simulink library "Contact_Forces_Lib"  (R2025a)
settings: Solver=ode45  StartTime=0.0  StopTime=10.0  RelTol=1e-3  EnableMultiTasking=on
undefined symbols (not defined in the file or in its folder): b_contact, custom_param_1, custom_param_2, Extr_Data_Ring, k_contact, l_cone, length_cylinder, length_tube, mu_kinetic, mu_static, pen_exponent, pen_full_damp_F, rad_s_cone, radius_cylinder, radius_tube, v_thr, X, Y, Z
libraries: nesl_utility x197, sm_lib x115, $bdroot x72, simulink x20, fl_lib x4
(part 8 of 12)

== system Contact_Forces_Lib/3D/Sphere to Tube Force Enabled/Demux ==
  Frc : Inport
  Demux : Demux  Outputs=8
  Demux1 : Demux  Outputs=3
  Scope : Scope  NumInputPorts=6
      settings: ActiveDisplayYMinimum=-4577.1518  ActiveDisplayYMaximum=26358.32622
  Simulink-PS Converter{,1..7} (8 alike) : nesl_utility/Simulink-PS Converter  PhysicalDomain=network_engine_domain  SubClassName=ps_input  LeftPortType=input  RightPortType=output  PseudoPeriodic=off  Frequencies=[]  NoiseDistribution=none  NoiseParameters=[]  Unit=1  AffineConversion=off  FilteringAndDerivatives=zero  SimscapeFilterOrder=1  InputFilterTimeConstant=0.005  UdotUserProvided=1
  FxF : PMIOPort  Side=Right
  FyF : PMIOPort  Port=2  Side=Right
  FzF : PMIOPort  Port=3  Side=Right
  TF : PMIOPort  Port=4  Side=Right
  FxB : PMIOPort  Port=5  Side=Right
  FyB : PMIOPort  Port=6  Side=Right
  FzB : PMIOPort  Port=7  Side=Right
  TB : PMIOPort  Port=8  Side=Right
  wires:
  Demux1/3 -> Scope/6  "Tz"
  Demux1/2 -> Scope/5  "Ty"
  Demux1/1 -> Scope/4  "Tx"
  Demux/5 -> Simulink-PS Converter3/1, Scope/1  "Fx"
  Demux/6 -> Simulink-PS Converter4/1, Scope/2  "Fy"
  Demux/8 -> Simulink-PS Converter5/1, Demux1/1
  Demux/7 -> Simulink-PS Converter7/1, Scope/3  "Fz"
  Demux/3 -> Simulink-PS Converter6/1  "Fz"
  Demux/4 -> Simulink-PS Converter2/1
  Demux/2 -> Simulink-PS Converter1/1  "Fy"
  Demux/1 -> Simulink-PS Converter/1  "Fx"
  Frc/1 -> Demux/1
  connections:
  Simulink-PS Converter7/RConn1 -- FzB/RConn1
  Simulink-PS Converter6/RConn1 -- FzF/RConn1
  Simulink-PS Converter1/RConn1 -- FyF/RConn1
  Simulink-PS Converter/RConn1 -- FxF/RConn1
  Simulink-PS Converter5/RConn1 -- TB/RConn1
  Simulink-PS Converter3/RConn1 -- FxB/RConn1
  Simulink-PS Converter4/RConn1 -- FyB/RConn1
  Simulink-PS Converter2/RConn1 -- TF/RConn1

== system Contact_Forces_Lib/3D/Sphere to Tube Force Enabled/Forces ==
  z : Inport
  rad : Inport  Port=2
  vrad : Inport  Port=3
  azm : Inport  Port=4
  vazm : Inport  Port=5
  wzf : Inport  Port=6
  R : Inport  Port=7
  vzf : Inport  Port=8
  wxf : Inport  Port=9
  wyf : Inport  Port=10
  Action Port : ActionPort
  Bus Creator : BusCreator  Inputs=6
  Calculate Penetration : Subsystem
  Ff : Subsystem
  Fn : Subsystem
  Force Law : $bdroot/Force Law  SystemSampleTime=-1  LabelModeActiveChoice=Linear  VariantActivationTime=update diagram  EmptyChoice=off  PassThrough=off  PassThroughVariantControl=(default)  EmptyChoiceVariantControl=(default)  AllowFlexibleInterface=on  Latency=0  AutoFrameSizeCalculation=off
  Gain : Gain  Gain=-1
  Mux : Mux  Inputs=8
  Product : Product
  Sum : Subsystem
  Sum1 : Sum  Inputs=+-
  Frc : Outport  VectorParamsAs1DForOutWhenUnconnected=off
  Out : Outport  Port=2  InitialOutput=[0]  VectorParamsAs1DForOutWhenUnconnected=off
  wires:
  wyf/1 -> Ff/11(wyf)
  wxf/1 -> Ff/10(wxf)
  Gain/1 -> Ff/1(Fn)
  vzf/1 -> Ff/9(vzf)
  wzf/1 -> Ff/6(wzf)
  vazm/1 -> Ff/5(vazm)
  Sum/8(TB) -> Mux/8
  Sum/7(FzB) -> Mux/7
  Ff/9(Ff) -> Bus Creator/6  "Friction Force"
  Sum/3(FzF) -> Mux/3
  Sum/6(FyB) -> Mux/6
  Sum/5(FxB) -> Mux/5
  Sum/4(TzF) -> Mux/4
  Mux/1 -> Frc/1
  Sum/1(FxF) -> Mux/1
  Sum/2(FyF) -> Mux/2
  azm/1 -> Ff/4(azm), Fn/4(azm)
  R/1 -> Ff/3(R), Fn/3(R)
  Sum1/1 -> Product/2
  Force Law/2 -> Sum1/2, Bus Creator/3  "Damp Force"
  Calculate Penetration/1(sign) -> Product/1
  Calculate Penetration/2(Pen) -> Force Law/1, Bus Creator/2, Ff/7(Pen)  "Penetration"
  Product/1 -> Gain/1, Fn/1(Fn), Bus Creator/5  "Normal Force"
  rad/1 -> Calculate Penetration/1(rad), Ff/8(rad)
  vrad/1 -> Calculate Penetration/2(vrad)
  Calculate Penetration/3(Pen Vel) -> Force Law/2, Bus Creator/1  "Penetration Vel"
  Force Law/1 -> Sum1/1, Bus Creator/4  "Spr Force"
  Bus Creator/1 -> Out/1
  z/1 -> Fn/2(z), Ff/2(z)
  Fn/2(FySphF) -> Sum/2(FnySphF)
  Fn/1(FxSphF) -> Sum/1(FnxSphF)
  Fn/3(FZSphF) -> Sum/3(FnzSphF)
  Fn/4(FxTubB) -> Sum/4(FnxTubB)
  Fn/5(FyTubB) -> Sum/5(FnyTubB)
  Fn/6(TxTubB) -> Sum/6(TnxTubB)
  Fn/7(TyTubB) -> Sum/7(TnyTubB)
  Ff/1(FxSphF) -> Sum/8(FfxSphF)
  Ff/2(FySohF) -> Sum/9(FfySphF)
  Ff/3(FzSphF) -> Sum/10(FfzSphF)
  Ff/4(FxTubB) -> Sum/11(FfxTubB)
  Ff/5(FyTubB) -> Sum/12(FfyTubB)
  Ff/6(FzTubB) -> Sum/13(FfzTubB)
  Ff/7(TSphF) -> Sum/14(TzSphF)
  Ff/8(TTubB) -> Sum/15(TTubB)

== system Contact_Forces_Lib/3D/Sphere to Tube Force Enabled/No Force ==
  Action Port : ActionPort
  Zeros : Constant  Value=[0 0 0 0 0 0 0 0 0 0 0 0]  SampleTime=0
  F : Outport  InitialOutput=[0]  VectorParamsAs1DForOutWhenUnconnected=off
  wires:
  Zeros/1 -> F/1

== system Contact_Forces_Lib/3D/Sphere to Tube Force Enabled/Sensing ==
  In : Inport
  Bus Selector : BusSelector  OutputSignals=wz
  In or Out : Subsystem
  PS-Simulink Converter{1..4,6..11} (10 alike) : nesl_utility/PS-Simulink Converter  PhysicalDomain=network_engine_domain  SubClassName=ps_output  LeftPortType=input  RightPortType=output  PseudoPeriodic=off  Frequencies=[]  VectorFormat=1-D array  Unit=1  AffineConversion=off
  Product : Product
  Rotation F in B : Gain  Gain=1/radius_sphere
  Sum : Sum  Inputs=|+-
  Transform Sensor Base : sm_lib/Frames and Transforms/Transform Sensor  MeasurementFrame=Base  RotationSequence=XYX  SenseAngle=off  SenseAxis=off  SenseQ=off  SenseR=on  SenseRotationSequence=off  SenseOmegaX=on  SenseOmegaY=on  SenseOmegaZ=on  SenseOmega=off  SenseQDot=off  SenseRDot=off  SenseRotationSequenceDot=off  SenseAlphaX=off  SenseAlphaY=off  SenseAlphaZ=off  SenseAlpha=off  SenseQDDot=off  SenseRDDot=off  SenseX=on  SenseY=on  SenseZ=on  SenseXYZ=off  SenseRad=off  SenseAzim=off  SenseDist=off  SenseInc=off  SenseXDot=on  SenseYDot=on  SenseZDot=on  SenseXYZDot=off  SenseRadDot=off  SenseAzimDot=off  SenseDistDot=off  SenseIncDot=off  SenseXDDot=off  SenseYDDot=off  SenseZDDot=off  SenseXYZDDot=off  SenseRadDDot=off  SenseAzimDDot=off  SenseDistDDot=off  SenseIncDDot=off
  rad_azm_cal : Subsystem
  F : PMIOPort  Side=Left
  B : PMIOPort  Port=2  Side=Left
  z : Outport  VectorParamsAs1DForOutWhenUnconnected=off
  rad : Outport  Port=2  VectorParamsAs1DForOutWhenUnconnected=off
  vrad : Outport  Port=3  VectorParamsAs1DForOutWhenUnconnected=off
  azm : Outport  Port=4  VectorParamsAs1DForOutWhenUnconnected=off
  vazm : Outport  Port=5  VectorParamsAs1DForOutWhenUnconnected=off
  wzf : Outport  Port=6  VectorParamsAs1DForOutWhenUnconnected=off
  R : Outport  Port=7  VectorParamsAs1DForOutWhenUnconnected=off
  vzf : Outport  Port=8  VectorParamsAs1DForOutWhenUnconnected=off
  wxf : Outport  Port=9  VectorParamsAs1DForOutWhenUnconnected=off
  wyf : Outport  Port=10  VectorParamsAs1DForOutWhenUnconnected=off
  wires:
  Sum/1 -> wzf/1
  rad_azm_cal/1(rad) -> In or Out/1(rad), rad/1
  Bus Selector/1 -> Rotation F in B/1  "<wz>"
  Product/1 -> Sum/2
  In/1 -> Bus Selector/1
  PS-Simulink Converter4/1 -> wyf/1
  PS-Simulink Converter3/1 -> wxf/1
  PS-Simulink Converter2/1 -> Sum/1
  PS-Simulink Converter1/1 -> vzf/1
  PS-Simulink Converter6/1 -> R/1
  rad_azm_cal/4(azmv) -> vazm/1
  rad_azm_cal/3(radv) -> vrad/1
  rad_azm_cal/2(azm) -> azm/1
  PS-Simulink Converter11/1 -> rad_azm_cal/4(Ydot)
  PS-Simulink Converter10/1 -> rad_azm_cal/3(Xdot)
  PS-Simulink Converter9/1 -> rad_azm_cal/2(Y)
  PS-Simulink Converter8/1 -> rad_azm_cal/1(X)
  PS-Simulink Converter7/1 -> z/1
  In or Out/1(factor) -> Product/2
  Rotation F in B/1 -> Product/1
  connections:
  PS-Simulink Converter2/LConn1 -- Transform Sensor Base/RConn5
  PS-Simulink Converter4/LConn1 -- Transform Sensor Base/RConn4
  Transform Sensor Base/RConn11 -- PS-Simulink Converter1/LConn1
  Transform Sensor Base/RConn10 -- PS-Simulink Converter11/LConn1
  Transform Sensor Base/RConn9 -- PS-Simulink Converter10/LConn1
  Transform Sensor Base/RConn8 -- PS-Simulink Converter7/LConn1
  Transform Sensor Base/RConn7 -- PS-Simulink Converter9/LConn1
  PS-Simulink Converter8/LConn1 -- Transform Sensor Base/RConn6
  PS-Simulink Converter3/LConn1 -- Transform Sensor Base/RConn3
  PS-Simulink Converter6/LConn1 -- Transform Sensor Base/RConn2
  Transform Sensor Base/LConn1 -- B/RConn1
  Transform Sensor Base/RConn1 -- F/RConn1

== system Contact_Forces_Lib/3D/Sphere to Tube Force Enabled/Set Output ==
  Frc : Inport
  En : Inport  Port=2
  FrameSep : Inport  Port=3
  Bus Creator : BusCreator  Inputs=7
  Bus Selector : BusSelector  OutputSignals=Normal Force,Friction Force,Penetration,Penetration Vel,Spr Force,Damp Force
  Demux : Demux  Outputs=6
  Mux : Mux  Inputs=6
  Product : Product
  Out : Outport  VectorParamsAs1DForOutWhenUnconnected=off
  wires:
  Bus Selector/2 -> Mux/2  "<Friction Force>"
  Bus Selector/4 -> Mux/4  "<Penetration Vel>"
  Bus Selector/6 -> Mux/6  "<Damp Force>"
  Bus Selector/3 -> Mux/3  "<Penetration>"
  Bus Creator/1 -> Out/1
  Bus Selector/1 -> Mux/1  "<Normal Force>"
  Bus Selector/5 -> Mux/5  "<Spr Force>"
  Frc/1 -> Bus Selector/1
  FrameSep/1 -> Bus Creator/7
  Mux/1 -> Product/2
  En/1 -> Product/1
  Product/1 -> Demux/1
  Demux/1 -> Bus Creator/1  "Normal Force"
  Demux/2 -> Bus Creator/2  "Friction Force"
  Demux/4 -> Bus Creator/4  "Penetration Vel"
  Demux/5 -> Bus Creator/5  "Spr Force"
  Demux/6 -> Bus Creator/6  "Damp Force"
  Demux/3 -> Bus Creator/3  "Penetration"

== system Contact_Forces_Lib/Force Law/Nonlinear/Smoothstep ==
  In1 : Inport
  Clamp : Saturate  UpperLimit=step_finish  LowerLimit=step_start
  Constant : Constant  Value=3
  Divide : Product  Inputs=*/
  Divide1 : Product  Inputs=****
  Gain : Gain  Gain=2
  Subtract : Sum  Inputs=+-
  Subtract1 : Sum  Inputs=-+
  Subtract2 : Sum
  Subtract3 : Sum  Inputs=+-
  Subtract4 : Sum  Inputs=+-
  max out : Constant  Value=max_out
  min out : Constant  Value=min_out
  step finish : Constant  Value=step_finish
  step start : Constant  Value=step_start
  Out1 : Outport  VectorParamsAs1DForOutWhenUnconnected=off
  wires:
  Subtract3/1 -> Divide1/4
  Subtract4/1 -> Divide1/1
  Gain/1 -> Subtract4/2
  Divide1/1 -> Subtract2/1
  step finish/1 -> Subtract1/2
  Clamp/1 -> Subtract/1
  max out/1 -> Subtract3/1
  min out/1 -> Subtract3/2, Subtract2/2
  Constant/1 -> Subtract4/1
  Subtract2/1 -> Out1/1
  Subtract/1 -> Divide/1
  Divide/1 -> Divide1/3, Divide1/2, Gain/1
  Subtract1/1 -> Divide/2
  In1/1 -> Clamp/1
  step start/1 -> Subtract/2, Subtract1/1

== system Contact_Forces_Lib/Friction Utilities/Stick-Slip Friction 1D/Lag Filter ==
  In : Inport
  Gain : Gain  Gain=1/b
  Integrator : Integrator  InitialCondition=x_initial
  Sum : Sum  Inputs=|+-  InputSameDT=on  SaturateOnIntegerOverflow=on  OutDataTypeStr=Inherit: Same as first input
  Out : Outport  VectorParamsAs1DForOutWhenUnconnected=off
  wires:
  Gain/1 -> Out/1, Sum/2
  Integrator/1 -> Gain/1
  In/1 -> Sum/1
  Sum/1 -> Integrator/1

== system Contact_Forces_Lib/Friction Utilities/Utilities/Product ==
  note: 1) Only subsystems can be added as variant choices at this level
      | 2) Blocks cannot be connected at this level as connectivity is
      | automatically determined at simulation, based on the active variant
  FcConst : Subsystem  VariantControl=FcConst
  FcVect : Subsystem  VariantControl=FcVect
  Fc : PMIOPort  Side=Right
  v : PMIOPort  Port=2  Side=Right

== system Contact_Forces_Lib/2D/Circle to Circle Force/Ff/Calculate vRel at CP  ==
  rad : Inport
  Pen : Inport  Port=2
  wz : Inport  Port=3
  vazm : Inport  Port=4
  Follower Radius : Constant  Value=cirF_rad
  Midpt Pen : Gain  Gain=0.5
  Product5 : Product
  Product6 : Product
  Sum{3,5..7} (4 alike) : Sum  Inputs=+-
  vRelCP : Outport  VectorParamsAs1DForOutWhenUnconnected=off
  rCirFtoCP : Outport  Port=2  VectorParamsAs1DForOutWhenUnconnected=off
  rCirBtoCP : Outport  Port=3  VectorParamsAs1DForOutWhenUnconnected=off
  wires:
  Follower Radius/1 -> Sum3/1
  Midpt Pen/1 -> Sum3/2
  Pen/1 -> Midpt Pen/1
  rad/1 -> Sum5/1
  Sum3/1 -> rCirFtoCP/1, Sum5/2, Product6/2
  vazm/1 -> Product5/1, Sum6/2
  Sum5/1 -> rCirBtoCP/1, Product5/2
  wz/1 -> Sum6/1
  Sum6/1 -> Product6/1
  Product5/1 -> Sum7/1
  Product6/1 -> Sum7/2
  Sum7/1 -> vRelCP/1

== system Contact_Forces_Lib/2D/Circle to Circle Force/Ff/Resolve Ff ==
  note: Resolve Friction Force in
      | Circle F reference frame
  note: Resolve Friction Force in
      | Circle B reference frame
  Ff : Inport
  R : Inport  Port=2
  azm : Inport  Port=3
  rCirFtoCP : Inport  Port=4
  rCirBtoCP : Inport  Port=5
  Ff in CirB : Subsystem
  Ff in CirF : Subsystem
  Tz : Subsystem
  FxCirB : Outport  VectorParamsAs1DForOutWhenUnconnected=off
  FyCirB : Outport  Port=2  VectorParamsAs1DForOutWhenUnconnected=off
  FyCirF : Outport  Port=3  VectorParamsAs1DForOutWhenUnconnected=off
  FxCirF : Outport  Port=4  VectorParamsAs1DForOutWhenUnconnected=off
  TzCirF : Outport  Port=5  VectorParamsAs1DForOutWhenUnconnected=off
  TzCirB : Outport  Port=6  VectorParamsAs1DForOutWhenUnconnected=off
  wires:
  Ff in CirF/2(FxCirF) -> FxCirF/1
  Ff in CirF/1(FyCirF) -> FyCirF/1
  R/1 -> Ff in CirF/1(R)
  azm/1 -> Ff in CirB/2(azm)
  Ff in CirB/2(FyCirB) -> Ff in CirF/3(FyCirB), FyCirB/1
  Ff in CirB/1(FxCirB) -> Ff in CirF/2(FxCirB), FxCirB/1
  Tz/2(TzF) -> TzCirF/1
  Tz/1(TzB) -> TzCirB/1
  Ff/1 -> Ff in CirB/1(Ff), Tz/3(Ff)
  rCirFtoCP/1 -> Tz/1(rCirFtoCP)
  rCirBtoCP/1 -> Tz/2(rCirBtoCP)

== system Contact_Forces_Lib/2D/Circle to Circle Force/Fn/Fn in CirB ==
  Fn : Inport
  azm : Inport  Port=2
  Divide1 : Product  Inputs=**
  Divide2 : Product  Inputs=**
  Gain2 : Gain  Gain=-1
  cos : Trigonometry  Operator=cos
  deg2rad : Gain  Gain=pi/180
  sin : Trigonometry
  FxCirB : Outport  VectorParamsAs1DForOutWhenUnconnected=off
  FyCirB : Outport  Port=2  VectorParamsAs1DForOutWhenUnconnected=off
  wires:
  azm/1 -> deg2rad/1
  Fn/1 -> Gain2/1
  Divide2/1 -> FyCirB/1  "Fy Cir"
  Divide1/1 -> FxCirB/1
  cos/1 -> Divide1/2
  sin/1 -> Divide2/2
  deg2rad/1 -> sin/1, cos/1
  Gain2/1 -> Divide2/1, Divide1/1

== system Contact_Forces_Lib/2D/Circle to Circle Force/Fn/Fn in CirF ==
  R : Inport
  FxCirB : Inport  Port=2
  FyCirB : Inport  Port=3
  Demux : Demux  Outputs=2
  Divide3 : Product  Inputs=**  Multiplication=Matrix(*)
  Gain : Gain  Gain=-1
  Mux1 : Mux  Inputs=2
  FyCirF : Outport  VectorParamsAs1DForOutWhenUnconnected=off
  FxCirF : Outport  Port=2  VectorParamsAs1DForOutWhenUnconnected=off
  wires:
  FxCirB/1 -> Mux1/2
  FyCirB/1 -> Mux1/1
  R/1 -> Divide3/1
  Divide3/1 -> Gain/1
  Mux1/1 -> Divide3/2
  Gain/1 -> Demux/1
  Demux/1 -> FyCirF/1
  Demux/2 -> FxCirF/1

== system Contact_Forces_Lib/2D/Circle to Circle Force Enabled/Ff/Calculate vRel at CP  ==
  rad : Inport
  Pen : Inport  Port=2
  wz : Inport  Port=3
  vazm : Inport  Port=4
  Follower Radius : Constant  Value=cirF_rad
  Midpt Pen : Gain  Gain=0.5
  Product5 : Product
  Product6 : Product
  Sum{3,5..7} (4 alike) : Sum  Inputs=+-
  vRelCP : Outport  VectorParamsAs1DForOutWhenUnconnected=off
  rCirFtoCP : Outport  Port=2  VectorParamsAs1DForOutWhenUnconnected=off
  rCirBtoCP : Outport  Port=3  VectorParamsAs1DForOutWhenUnconnected=off
  wires:
  Sum7/1 -> vRelCP/1
  Product6/1 -> Sum7/2
  Product5/1 -> Sum7/1
  Sum6/1 -> Product6/1
  wz/1 -> Sum6/1
  Sum5/1 -> Product5/2, rCirBtoCP/1
  vazm/1 -> Sum6/2, Product5/1
  Sum3/1 -> Product6/2, Sum5/2, rCirFtoCP/1
  rad/1 -> Sum5/1
  Pen/1 -> Midpt Pen/1
  Midpt Pen/1 -> Sum3/2
  Follower Radius/1 -> Sum3/1

== system Contact_Forces_Lib/2D/Circle to Circle Force Enabled/Ff/Resolve Ff ==
  note: Resolve Friction Force in
      | Circle B reference frame
  note: Resolve Friction Force in
      | Circle F reference frame
  Ff : Inport
  R : Inport  Port=2
  azm : Inport  Port=3
  rCirFtoCP : Inport  Port=4
  rCirBtoCP : Inport  Port=5
  Ff in CirB : Subsystem
  Ff in CirF : Subsystem
  Tz : Subsystem
  FxCirB : Outport  VectorParamsAs1DForOutWhenUnconnected=off
  FyCirB : Outport  Port=2  VectorParamsAs1DForOutWhenUnconnected=off
  FyCirF : Outport  Port=3  VectorParamsAs1DForOutWhenUnconnected=off
  FxCirF : Outport  Port=4  VectorParamsAs1DForOutWhenUnconnected=off
  TzCirF : Outport  Port=5  VectorParamsAs1DForOutWhenUnconnected=off
  TzCirB : Outport  Port=6  VectorParamsAs1DForOutWhenUnconnected=off
  wires:
  rCirBtoCP/1 -> Tz/2(rCirBtoCP)
  rCirFtoCP/1 -> Tz/1(rCirFtoCP)
  Ff/1 -> Tz/3(Ff), Ff in CirB/1(Ff)
  Tz/1(TzB) -> TzCirB/1
  Tz/2(TzF) -> TzCirF/1
  Ff in CirB/1(FxCirB) -> FxCirB/1, Ff in CirF/2(FxCirB)
  Ff in CirB/2(FyCirB) -> FyCirB/1, Ff in CirF/3(FyCirB)
  azm/1 -> Ff in CirB/2(azm)
  R/1 -> Ff in CirF/1(R)
  Ff in CirF/1(FyCirF) -> FyCirF/1
  Ff in CirF/2(FxCirF) -> FxCirF/1

== system Contact_Forces_Lib/2D/Circle to Circle Force Enabled/Fn/Fn in CirB ==
  Fn : Inport
  azm : Inport  Port=2
  Divide1 : Product  Inputs=**
  Divide2 : Product  Inputs=**
  Gain2 : Gain  Gain=-1
  cos : Trigonometry  Operator=cos
  deg2rad : Gain  Gain=pi/180
  sin : Trigonometry
  FxCirB : Outport  VectorParamsAs1DForOutWhenUnconnected=off
  FyCirB : Outport  Port=2  VectorParamsAs1DForOutWhenUnconnected=off
  wires:
  Gain2/1 -> Divide1/1, Divide2/1
  deg2rad/1 -> cos/1, sin/1
  sin/1 -> Divide2/2
  cos/1 -> Divide1/2
  Divide1/1 -> FxCirB/1
  Divide2/1 -> FyCirB/1  "Fy Cir"
  Fn/1 -> Gain2/1
  azm/1 -> deg2rad/1

== system Contact_Forces_Lib/2D/Circle to Circle Force Enabled/Fn/Fn in CirF ==
  R : Inport
  FxCirB : Inport  Port=2
  FyCirB : Inport  Port=3
  Demux : Demux  Outputs=2
  Divide3 : Product  Inputs=**  Multiplication=Matrix(*)
  Gain : Gain  Gain=-1
  Mux1 : Mux  Inputs=2
  FyCirF : Outport  VectorParamsAs1DForOutWhenUnconnected=off
  FxCirF : Outport  Port=2  VectorParamsAs1DForOutWhenUnconnected=off
  wires:
  Demux/2 -> FxCirF/1
  Demux/1 -> FyCirF/1
  Gain/1 -> Demux/1
  Mux1/1 -> Divide3/2
  Divide3/1 -> Gain/1
  R/1 -> Divide3/1
  FyCirB/1 -> Mux1/1
  FxCirB/1 -> Mux1/2

== system Contact_Forces_Lib/2D/Circle to Finite Line Force/Forces/Resolve Forces ==
  note: For circle, uses forces as calculated.
      | For line, force must be applied at CG.
      |        Apply torque corresponding to equivalent couple.
  Moment arm : Inport
  Pos Cmp : Inport  Port=2
  X Sep : Inport  Port=3
  Spr Force Mag : Inport  Port=4
  Damp Force Mag : Inport  Port=5
  Vel Cmp : Inport  Port=6
  Unit Vector : Inport  Port=7
  vy : Inport  Port=8
  wz : Inport  Port=9
  Divide4 : Product  Inputs=**
  FnCir : Subsystem
  FnLin : Subsystem
  Friction : Subsystem
  Gain : Gain  Gain=-1
  Product : Product  RndMeth=Zero
  Product1 : Product  RndMeth=Zero
  Sum{,1..4} (5 alike) : Sum
  Fx Cir : Outport  VectorParamsAs1DForOutWhenUnconnected=off
  Fy Cir : Outport  Port=2  VectorParamsAs1DForOutWhenUnconnected=off
  Tz Cir : Outport  Port=3  VectorParamsAs1DForOutWhenUnconnected=off
  Fx Lin : Outport  Port=4  VectorParamsAs1DForOutWhenUnconnected=off
  Fy Lin : Outport  Port=5  VectorParamsAs1DForOutWhenUnconnected=off
  Tz Lin : Outport  Port=6  VectorParamsAs1DForOutWhenUnconnected=off
  Fn : Outport  Port=7  VectorParamsAs1DForOutWhenUnconnected=off
  Ff : Outport  Port=8  VectorParamsAs1DForOutWhenUnconnected=off
  wires:
  X Sep/1 -> Friction/3(X Sep)
  Friction/5(TzCir) -> Tz Cir/1
  Sum1/1 -> Friction/2(Fn), FnCir/2(Fn), Divide4/1, Fn/1, FnLin/1(Fn)
  Sum2/1 -> Fx Cir/1
  Sum3/1 -> Fy Cir/1
  Sum4/1 -> Fy Lin/1
  FnLin/1(FxLin) -> Fx Lin/1
  Friction/3(FyLin) -> Sum4/1
  FnLin/2(FyLin) -> Sum4/2
  Friction/2(FyCir) -> Sum3/2
  FnCir/2(FyCir) -> Sum3/1
  FnCir/1(FxCir) -> Sum2/1
  Friction/1(FxCir) -> Sum2/2
  Friction/4(TzLin) -> Sum/1
  Sum/1 -> Tz Lin/1
  wz/1 -> Friction/5(wz)
  vy/1 -> Friction/4(vLin)
  Vel Cmp/1 -> Product1/1
  Pos Cmp/1 -> Product/1
  Unit Vector/1 -> Friction/1(Unit Vector), FnCir/1(Unit Vector)
  Gain/1 -> Sum/2  "Equivalent Couple"
  Divide4/1 -> Gain/1
  Moment arm/1 -> Divide4/2
  Product1/1 -> Sum1/2
  Damp Force Mag/1 -> Product1/2
  Spr Force Mag/1 -> Product/2
  Product/1 -> Sum1/1
  Friction/6(Ff) -> Ff/1

== system Contact_Forces_Lib/2D/Circle to Finite Line Force/Forces/Subsystem ==
  Fn : Inport
  Ff : Inport  Port=2
  Abs : Abs  ZeroCross=off  SaturateOnIntegerOverflow=off
  Add : Sum
  Constant : Constant  Value=0
  Mux1 : Mux  Inputs=2
  Out : Outport  VectorParamsAs1DForOutWhenUnconnected=off
  wires:
  Mux1/1 -> Add/1
  Fn/1 -> Abs/1
  Ff/1 -> Mux1/2
  Add/1 -> Out/1
  Constant/1 -> Add/2
  Abs/1 -> Mux1/1

== system Contact_Forces_Lib/2D/Circle to Finite Line Force Enabled/Forces/Resolve Forces ==
  note: For circle, uses forces as calculated.
      | For line, force must be applied at CG.
      |        Apply torque corresponding to equivalent couple.
  Moment arm : Inport
  Pos Cmp : Inport  Port=2
  X Sep : Inport  Port=3
  Spr Force Mag : Inport  Port=4
  Damp Force Mag : Inport  Port=5
  Vel Cmp : Inport  Port=6
  Unit Vector : Inport  Port=7
  vy : Inport  Port=8
  wz : Inport  Port=9
  Divide4 : Product  Inputs=**
  FnCir : Subsystem
  FnLin : Subsystem
  Friction : Subsystem
  Gain : Gain  Gain=-1
  Product : Product  RndMeth=Zero
  Product1 : Product  RndMeth=Zero
  Sum{,1..4} (5 alike) : Sum
  Fx Cir : Outport  VectorParamsAs1DForOutWhenUnconnected=off
  Fy Cir : Outport  Port=2  VectorParamsAs1DForOutWhenUnconnected=off
  Tz Cir : Outport  Port=3  VectorParamsAs1DForOutWhenUnconnected=off
  Fx Lin : Outport  Port=4  VectorParamsAs1DForOutWhenUnconnected=off
  Fy Lin : Outport  Port=5  VectorParamsAs1DForOutWhenUnconnected=off
  Tz Lin : Outport  Port=6  VectorParamsAs1DForOutWhenUnconnected=off
  Fn : Outport  Port=7  VectorParamsAs1DForOutWhenUnconnected=off
  Ff : Outport  Port=8  VectorParamsAs1DForOutWhenUnconnected=off
  wires:
  Friction/6(Ff) -> Ff/1
  Product/1 -> Sum1/1
  Spr Force Mag/1 -> Product/2
  Damp Force Mag/1 -> Product1/2
  Product1/1 -> Sum1/2
  Moment arm/1 -> Divide4/2
  Divide4/1 -> Gain/1
  Gain/1 -> Sum/2  "Equivalent Couple"
  Unit Vector/1 -> FnCir/1(Unit Vector), Friction/1(Unit Vector)
  Pos Cmp/1 -> Product/1
  Vel Cmp/1 -> Product1/1
  vy/1 -> Friction/4(vLin)
  wz/1 -> Friction/5(wz)
  Sum/1 -> Tz Lin/1
  Friction/4(TzLin) -> Sum/1
  Friction/1(FxCir) -> Sum2/2
  FnCir/1(FxCir) -> Sum2/1
  FnCir/2(FyCir) -> Sum3/1
  Friction/2(FyCir) -> Sum3/2
  FnLin/2(FyLin) -> Sum4/2
  Friction/3(FyLin) -> Sum4/1
  FnLin/1(FxLin) -> Fx Lin/1
  Sum4/1 -> Fy Lin/1
  Sum3/1 -> Fy Cir/1
  Sum2/1 -> Fx Cir/1
  Sum1/1 -> FnLin/1(Fn), Fn/1, Divide4/1, FnCir/2(Fn), Friction/2(Fn)
  Friction/5(TzCir) -> Tz Cir/1
  X Sep/1 -> Friction/3(X Sep)

== system Contact_Forces_Lib/2D/Circle to Finite Line Force Enabled/Forces/Subsystem ==
  Fn : Inport
  Ff : Inport  Port=2
  Abs : Abs  ZeroCross=off  SaturateOnIntegerOverflow=off
  Add : Sum
  Constant : Constant  Value=0
  Mux1 : Mux  Inputs=2
  Out : Outport  VectorParamsAs1DForOutWhenUnconnected=off
  wires:
  Abs/1 -> Mux1/1
  Constant/1 -> Add/2
  Add/1 -> Out/1
  Ff/1 -> Mux1/2
  Fn/1 -> Abs/1
  Mux1/1 -> Add/1

== system Contact_Forces_Lib/2D/Circle to Ring Force/Forces/Calculate Penetration ==
  note: Calculates CirF frame to midpoint of ring wall.
      | Absolute value makes it valid for inside or outside contact.
      | Noting the sign allows us to apply the force correctly
  rad : Inport
  vrad : Inport  Port=2
  Abs : Abs  ZeroCross=off  SaturateOnIntegerOverflow=off
  Constant : Constant  Value=radius_circle+d_ring/2
  Dead Zone : DeadZone  LowerValue=-inf  UpperValue=0
  Product : Product
  Sign : Signum  ZeroCross=off
  Sum : Sum  Inputs=+-
  Sum1 : Sum  Inputs=+-
  radius ring : Constant  Value=radius_ring
  sign : Outport  VectorParamsAs1DForOutWhenUnconnected=off
  Pen : Outport  Port=2  VectorParamsAs1DForOutWhenUnconnected=off
  Pen Vel : Outport  Port=3  VectorParamsAs1DForOutWhenUnconnected=off
  wires:
  radius ring/1 -> Sum1/1
  Sum1/1 -> Sign/1, Abs/1
  rad/1 -> Sum1/2
  Abs/1 -> Sum/2
  Sign/1 -> Product/1, sign/1
  Product/1 -> Pen Vel/1
  vrad/1 -> Product/2
  Sum/1 -> Dead Zone/1
  Constant/1 -> Sum/1
  Dead Zone/1 -> Pen/1

== system Contact_Forces_Lib/2D/Circle to Ring Force/Forces/Ff ==
  R : Inport
  azm : Inport  Port=2
  vazm : Inport  Port=3
  wzf : Inport  Port=4
  Fn : Inport  Port=5
  Pen : Inport  Port=6
  rad : Inport  Port=7
  "Calculate vRel at CP " : Subsystem
  Friction Law : $bdroot/Friction Law  SystemSampleTime=-1  LabelModeActiveChoice=Stick_Slip_C  VariantActivationTime=update diagram  EmptyChoice=off  PassThrough=off  PassThroughVariantControl=(default)  EmptyChoiceVariantControl=(default)  AllowFlexibleInterface=on  Latency=0  AutoFrameSizeCalculation=off
  Resolve Ff : Subsystem
  Sign : Signum  ZeroCross=off
  FxCirF : Outport  VectorParamsAs1DForOutWhenUnconnected=off
  FyCirF : Outport  Port=2  VectorParamsAs1DForOutWhenUnconnected=off
  FxCirB : Outport  Port=3  VectorParamsAs1DForOutWhenUnconnected=off
  FyCirB : Outport  Port=4  VectorParamsAs1DForOutWhenUnconnected=off
  TzCirF : Outport  Port=5  VectorParamsAs1DForOutWhenUnconnected=off
  TzCirB : Outport  Port=6  VectorParamsAs1DForOutWhenUnconnected=off
  Ff : Outport  Port=7  VectorParamsAs1DForOutWhenUnconnected=off
  wires:
  Resolve Ff/6(TzRinB) -> TzCirB/1
  Resolve Ff/3(TzCirF) -> TzCirF/1
  Resolve Ff/5(FyRinB) -> FyCirB/1
  Resolve Ff/4(FxRinB) -> FxCirB/1
  Resolve Ff/2(FyCirF) -> FyCirF/1
  Resolve Ff/1(FxCirF) -> FxCirF/1
  Friction Law/1 -> Resolve Ff/2(Ff), Ff/1
  "Calculate vRel at CP "/1(vRelCP) -> Friction Law/2
  wzf/1 -> "Calculate vRel at CP "/5(wzf)
  vazm/1 -> "Calculate vRel at CP "/4(vazm)
  rad/1 -> "Calculate vRel at CP "/2(rad)
  Fn/1 -> Sign/1, Friction Law/1
  Pen/1 -> "Calculate vRel at CP "/3(Pen)
  azm/1 -> Resolve Ff/4(azm)
  R/1 -> Resolve Ff/3(R)
  "Calculate vRel at CP "/2(rCirFtoCP) -> Resolve Ff/5(rCirFtoCP)
  "Calculate vRel at CP "/3(rRinBtoCP) -> Resolve Ff/6(rRinBtoCP)
  Sign/1 -> [InOut]
  [InOut] -> "Calculate vRel at CP "/1(InOut)
  [InOut] -> Resolve Ff/1(Fn)

== system Contact_Forces_Lib/2D/Circle to Ring Force/Forces/Fn ==
  note: Resolve Normal Force in
      | Circle B reference frame
  note: Resolve Normal Force in
      | Circle F reference frame
  Fn : Inport
  R : Inport  Port=2
  azm : Inport  Port=3
  Fn in CirB : Subsystem
  Fn in CirF : Subsystem
  FxCirF : Outport  VectorParamsAs1DForOutWhenUnconnected=off
  FyCirF : Outport  Port=2  VectorParamsAs1DForOutWhenUnconnected=off
  FxCirB : Outport  Port=3  VectorParamsAs1DForOutWhenUnconnected=off
  FyCirB : Outport  Port=4  VectorParamsAs1DForOutWhenUnconnected=off
  wires:
  Fn in CirF/1(FyCirF) -> FyCirF/1
  Fn in CirB/1(FxCirB) -> FxCirB/1, Fn in CirF/2(FxCirB)
  Fn in CirB/2(FyCirB) -> Fn in CirF/3(FyCirB), FyCirB/1
  Fn/1 -> Fn in CirB/1(Fn)
  azm/1 -> Fn in CirB/2(azm)
  R/1 -> Fn in CirF/1(R)
  Fn in CirF/2(FxCirF) -> FxCirF/1

== system Contact_Forces_Lib/2D/Circle to Ring Force/Forces/Sum ==
  FnxCirF : Inport
  FnyCirF : Inport  Port=2
  FnxCirB : Inport  Port=3
  FnyCirB : Inport  Port=4
  FfxCirF : Inport  Port=5
  FfyCirF : Inport  Port=6
  FfxCirB : Inport  Port=7
  FfyCirB : Inport  Port=8
  TzCirF : Inport  Port=9
  TzCirB : Inport  Port=10
  Sum{2..5} (4 alike) : Sum
  FxF : Outport  VectorParamsAs1DForOutWhenUnconnected=off
  FyF : Outport  Port=2  VectorParamsAs1DForOutWhenUnconnected=off
  TzF : Outport  Port=3  VectorParamsAs1DForOutWhenUnconnected=off
  FxB : Outport  Port=4  VectorParamsAs1DForOutWhenUnconnected=off
  FyB : Outport  Port=5  VectorParamsAs1DForOutWhenUnconnected=off
  TzB : Outport  Port=6  VectorParamsAs1DForOutWhenUnconnected=off
  wires:
  TzCirF/1 -> TzF/1
  TzCirB/1 -> TzB/1
  FfyCirB/1 -> Sum5/2
  FfxCirB/1 -> Sum3/2
  FfyCirF/1 -> Sum2/2
  FfxCirF/1 -> Sum4/2
  Sum5/1 -> FyB/1
  Sum3/1 -> FxB/1
  Sum2/1 -> FyF/1
  Sum4/1 -> FxF/1
  FnyCirB/1 -> Sum5/1
  FnxCirB/1 -> Sum3/1
  FnyCirF/1 -> Sum2/1
  FnxCirF/1 -> Sum4/1

== system Contact_Forces_Lib/2D/Composite Forces/Box to Belt Force/Belt Ends ==
  In : Inport
  Add1 : Sum  Inputs=++++
  Circle to Finite Line E1 Front : $bdroot/2D/Circle to Finite Line Force Enabled  circle_rad=belt_h/2  line_depth=box_h/2  line_length=box_l  force_law=Linear  k_contact=k_contact_box2belt  b_contact=b_contact_box2belt  pen_full_damp_F=pen_full_damp_F_box2belt  pen_exponent=pen_exponent_box2belt  custom_param_1=1  custom_param_2=1  friction_law=Stick-Slip Continuous  mu_kinetic=mu_kinetic_box2belt  mu_static=mu_static_box2belt  v_thr=v_thr_box2belt  vis_on=off  vis_opc_en=0  vis_len_linBz=vis_len_boxz  vis_len_linBx=vis_len_boxx  vis_len_cirFz=vis_len_beltz  vis_len_cirFx=vis_len_beltx  vis_clr=vis_clr_box2belt  vis_opc=vis_opc_box2belt
  Circle to Finite Line E1 Top : $bdroot/2D/Circle to Finite Line Force Enabled  circle_rad=belt_h/2  line_depth=box_l/2  line_length=box_h  force_law=Linear  k_contact=k_contact_box2belt  b_contact=b_contact_box2belt  pen_full_damp_F=pen_full_damp_F_box2belt  pen_exponent=pen_exponent_box2belt  custom_param_1=1  custom_param_2=1  friction_law=Stick-Slip Continuous  mu_kinetic=mu_kinetic_box2belt  mu_static=mu_static_box2belt  v_thr=v_thr_box2belt  vis_on=off  vis_opc_en=0  vis_len_linBz=vis_len_boxz  vis_len_linBx=vis_len_boxx  vis_len_cirFz=vis_len_beltz  vis_len_cirFx=vis_len_beltx  vis_clr=vis_clr_box2belt  vis_opc=vis_opc_box2belt
  Circle to Finite Line E2 Front : $bdroot/2D/Circle to Finite Line Force Enabled  circle_rad=belt_h/2  line_depth=box_h/2  line_length=box_l  force_law=Linear  k_contact=k_contact_box2belt  b_contact=b_contact_box2belt  pen_full_damp_F=pen_full_damp_F_box2belt  pen_exponent=pen_exponent_box2belt  custom_param_1=1  custom_param_2=1  friction_law=Stick-Slip Continuous  mu_kinetic=mu_kinetic_box2belt  mu_static=mu_static_box2belt  v_thr=v_thr_box2belt  vis_on=off  vis_opc_en=0  vis_len_linBz=vis_len_boxz  vis_len_linBx=vis_len_boxx  vis_len_cirFz=vis_len_beltz  vis_len_cirFx=vis_len_beltx  vis_clr=vis_clr_box2belt  vis_opc=vis_opc_box2belt
  Circle to Finite Line E2 Top : $bdroot/2D/Circle to Finite Line Force Enabled  circle_rad=belt_h/2  line_depth=box_l/2  line_length=box_h  force_law=Linear  k_contact=k_contact_box2belt  b_contact=b_contact_box2belt  pen_full_damp_F=pen_full_damp_F_box2belt  pen_exponent=pen_exponent_box2belt  custom_param_1=1  custom_param_2=1  friction_law=Stick-Slip Continuous  mu_kinetic=mu_kinetic_box2belt  mu_static=mu_static_box2belt  v_thr=v_thr_box2belt  vis_on=off  vis_opc_en=0  vis_len_linBz=vis_len_boxz  vis_len_linBx=vis_len_boxx  vis_len_cirFz=vis_len_beltz  vis_len_cirFx=vis_len_beltx  vis_clr=vis_clr_box2belt  vis_opc=vis_opc_box2belt
  Sensing C5 : Subsystem
  Sensing C6 : Subsystem
  Sensing C7 : Subsystem
  Sensing C8 : Subsystem
  Transform Box Front Back : sm_lib/Frames and Transforms/Rigid Transform  RotationMethod=StandardAxis  FollAlignAxisA=+X  BaseAlignAxisA=+Y  FollAlignAxisB=+Y  BaseAlignAxisB=+Z  RotationStandardAxis=+Z  RotationAngle=-90  RotationAngleUnits=deg  RotationArbitraryAxis=[0 0 1]  RotationSequenceAxes=FollowerAxes  RotationSequence=XYX  RotationSequenceAngles=[0 0 0]  RotationSequenceAnglesUnits=deg  RotationMatrix=[1 0 0; 0 1 0; 0 0 1]  Quaternion=[1 0 0 0]  TranslationMethod=Cartesian  TranslationCartesianOffset=[0 0 0]  TranslationCartesianOffsetUnits=m  TranslationStandardAxis=+Z  TranslationStandardOffset=0  TranslationStandardOffsetUnits=m  TranslationROffset=0  TranslationROffsetUnits=m  TranslationThetaOffset=0  TranslationThetaOffsetUnits=deg  TranslationZOffset=0  TranslationZOffsetUnits=m
  Transform End 1 : sm_lib/Frames and Transforms/Rigid Transform  RotationMethod=None  FollAlignAxisA=+X  BaseAlignAxisA=+Y  FollAlignAxisB=+Y  BaseAlignAxisB=+Z  RotationStandardAxis=+Z  RotationAngle=0  RotationAngleUnits=deg  RotationArbitraryAxis=[0 0 1]  RotationSequenceAxes=FollowerAxes  RotationSequence=XYX  RotationSequenceAngles=[0 0 0]  RotationSequenceAnglesUnits=deg  RotationMatrix=[1 0 0; 0 1 0; 0 0 1]  Quaternion=[1 0 0 0]  TranslationMethod=StandardAxis  TranslationCartesianOffset=[0 0 0]  TranslationCartesianOffsetUnits=m  TranslationStandardAxis=+Y  TranslationStandardOffset=belt_l/2  TranslationStandardOffsetUnits=m  TranslationROffset=0  TranslationROffsetUnits=m  TranslationThetaOffset=0  TranslationThetaOffsetUnits=deg  TranslationZOffset=0  TranslationZOffsetUnits=m
  Transform End 2 : sm_lib/Frames and Transforms/Rigid Transform  RotationMethod=None  FollAlignAxisA=+X  BaseAlignAxisA=+Y  FollAlignAxisB=+Y  BaseAlignAxisB=+Z  RotationStandardAxis=+Z  RotationAngle=0  RotationAngleUnits=deg  RotationArbitraryAxis=[0 0 1]  RotationSequenceAxes=FollowerAxes  RotationSequence=XYX  RotationSequenceAngles=[0 0 0]  RotationSequenceAnglesUnits=deg  RotationMatrix=[1 0 0; 0 1 0; 0 0 1]  Quaternion=[1 0 0 0]  TranslationMethod=StandardAxis  TranslationCartesianOffset=[0 0 0]  TranslationCartesianOffsetUnits=m  TranslationStandardAxis=-Y  TranslationStandardOffset=belt_l/2  TranslationStandardOffsetUnits=m  TranslationROffset=0  TranslationROffsetUnits=m  TranslationThetaOffset=0  TranslationThetaOffsetUnits=deg  TranslationZOffset=0  TranslationZOffsetUnits=m
  Box : PMIOPort  Side=Right
  Bel : PMIOPort  Port=2  Side=Left
  Fn : Outport  VectorParamsAs1DForOutWhenUnconnected=off
  wires:
  Circle to Finite Line E2 Top/1 -> Sensing C7/1(S)
  Sensing C7/1(Fn) -> Add1/1
  In/1 -> Circle to Finite Line E2 Top/1, Circle to Finite Line E2 Front/1, Circle to Finite Line E1 Top/1, Circle to Finite Line E1 Front/1
  Sensing C8/1(Fn) -> Add1/3
  Circle to Finite Line E1 Front/1 -> Sensing C6/1(S)
  Sensing C6/1(Fn) -> Add1/4
  Sensing C5/1(Fn) -> Add1/2
  Circle to Finite Line E2 Front/1 -> Sensing C5/1(S)
  Circle to Finite Line E1 Top/1 -> Sensing C8/1(S)
  Add1/1 -> Fn/1
  connections:
  Bel/RConn1 -- Transform End 1/LConn1 -- Transform End 2/LConn1
  Circle to Finite Line E1 Top/RConn1 -- Circle to Finite Line E2 Top/RConn1 -- Transform Box Front Back/LConn1 -- Box/RConn1
  Circle to Finite Line E1 Top/LConn1 -- Transform End 1/RConn1 -- Circle to Finite Line E1 Front/LConn1
  Transform Box Front Back/RConn1 -- Circle to Finite Line E2 Front/RConn1 -- Circle to Finite Line E1 Front/RConn1
  Circle to Finite Line E2 Front/LConn1 -- Circle to Finite Line E2 Top/LConn1 -- Transform End 2/RConn1

== system Contact_Forces_Lib/2D/Composite Forces/Box to Belt Force/Belt Faces ==
  In1 : Inport
  Add : Sum  Inputs=++++
  Circle to Finite Line Force C{1..4} (4 alike) : $bdroot/2D/Circle to Finite Line Force Enabled  circle_rad=contact_circle_rad_box2belt  line_depth=belt_h/2  line_length=belt_l  force_law=Linear  k_contact=k_contact_box2belt  b_contact=b_contact_box2belt  pen_full_damp_F=pen_full_damp_F_box2belt  pen_exponent=pen_exponent_box2belt  custom_param_1=1  custom_param_2=1  friction_law=Stick-Slip Continuous  mu_kinetic=mu_kinetic_box2belt  mu_static=mu_static_box2belt  v_thr=v_thr_box2belt  vis_on=off  vis_opc_en=0  vis_len_linBz=vis_len_beltz  vis_len_linBx=vis_len_beltx  vis_len_cirFz=vis_len_boxz  vis_len_cirFx=vis_len_boxx  vis_clr=vis_clr_box2belt  vis_opc=vis_opc_box2belt
  Sensing C1 : Subsystem
  Sensing C2 : Subsystem
  Sensing C3 : Subsystem
  Sensing C4 : Subsystem
  Transform C1 : sm_lib/Frames and Transforms/Rigid Transform  RotationMethod=None  FollAlignAxisA=+X  BaseAlignAxisA=+Y  FollAlignAxisB=+Y  BaseAlignAxisB=+Z  RotationStandardAxis=+Z  RotationAngle=0  RotationAngleUnits=deg  RotationArbitraryAxis=[0 0 1]  RotationSequenceAxes=FollowerAxes  RotationSequence=XYX  RotationSequenceAngles=[0 0 0]  RotationSequenceAnglesUnits=deg  RotationMatrix=[1 0 0; 0 1 0; 0 0 1]  Quaternion=[1 0 0 0]  TranslationMethod=Cartesian  TranslationCartesianOffset=[box_l/2-contact_circle_rad_box2belt -(box_h/2-contact_circle_rad_box2belt) 0]  TranslationCartesianOffsetUnits=m  TranslationStandardAxis=+Z  TranslationStandardOffset=0  TranslationStandardOffsetUnits=m  TranslationROffset=0  TranslationROffsetUnits=m  TranslationThetaOffset=0  TranslationThetaOffsetUnits=deg  TranslationZOffset=0  TranslationZOffsetUnits=m
  Transform C2 : sm_lib/Frames and Transforms/Rigid Transform  RotationMethod=None  FollAlignAxisA=+X  BaseAlignAxisA=+Y  FollAlignAxisB=+Y  BaseAlignAxisB=+Z  RotationStandardAxis=+Z  RotationAngle=0  RotationAngleUnits=deg  RotationArbitraryAxis=[0 0 1]  RotationSequenceAxes=FollowerAxes  RotationSequence=XYX  RotationSequenceAngles=[0 0 0]  RotationSequenceAnglesUnits=deg  RotationMatrix=[1 0 0; 0 1 0; 0 0 1]  Quaternion=[1 0 0 0]  TranslationMethod=Cartesian  TranslationCartesianOffset=[-(box_l/2-contact_circle_rad_box2belt) -(box_h/2-contact_circle_rad_box2belt) 0]  TranslationCartesianOffsetUnits=m  TranslationStandardAxis=+Z  TranslationStandardOffset=0  TranslationStandardOffsetUnits=m  TranslationROffset=0  TranslationROffsetUnits=m  TranslationThetaOffset=0  TranslationThetaOffsetUnits=deg  TranslationZOffset=0  TranslationZOffsetUnits=m
  Transform C3 : sm_lib/Frames and Transforms/Rigid Transform  RotationMethod=None  FollAlignAxisA=+X  BaseAlignAxisA=+Y  FollAlignAxisB=+Y  BaseAlignAxisB=+Z  RotationStandardAxis=+Z  RotationAngle=0  RotationAngleUnits=deg  RotationArbitraryAxis=[0 0 1]  RotationSequenceAxes=FollowerAxes  RotationSequence=XYX  RotationSequenceAngles=[0 0 0]  RotationSequenceAnglesUnits=deg  RotationMatrix=[1 0 0; 0 1 0; 0 0 1]  Quaternion=[1 0 0 0]  TranslationMethod=Cartesian  TranslationCartesianOffset=[box_l/2-contact_circle_rad_box2belt (box_h/2-contact_circle_rad_box2belt) 0]  TranslationCartesianOffsetUnits=m  TranslationStandardAxis=+Z  TranslationStandardOffset=0  TranslationStandardOffsetUnits=m  TranslationROffset=0  TranslationROffsetUnits=m  TranslationThetaOffset=0  TranslationThetaOffsetUnits=deg  TranslationZOffset=0  TranslationZOffsetUnits=m
  Transform C4 : sm_lib/Frames and Transforms/Rigid Transform  RotationMethod=None  FollAlignAxisA=+X  BaseAlignAxisA=+Y  FollAlignAxisB=+Y  BaseAlignAxisB=+Z  RotationStandardAxis=+Z  RotationAngle=0  RotationAngleUnits=deg  RotationArbitraryAxis=[0 0 1]  RotationSequenceAxes=FollowerAxes  RotationSequence=XYX  RotationSequenceAngles=[0 0 0]  RotationSequenceAnglesUnits=deg  RotationMatrix=[1 0 0; 0 1 0; 0 0 1]  Quaternion=[1 0 0 0]  TranslationMethod=Cartesian  TranslationCartesianOffset=[-(box_l/2-contact_circle_rad_box2belt) (box_h/2-contact_circle_rad_box2belt) 0]  TranslationCartesianOffsetUnits=m  TranslationStandardAxis=+Z  TranslationStandardOffset=0  TranslationStandardOffsetUnits=m  TranslationROffset=0  TranslationROffsetUnits=m  TranslationThetaOffset=0  TranslationThetaOffsetUnits=deg  TranslationZOffset=0  TranslationZOffsetUnits=m
  Box : PMIOPort  Side=Right
  Bel : PMIOPort  Port=2  Side=Left
  Fn : Outport  VectorParamsAs1DForOutWhenUnconnected=off
  wires:
  In1/1 -> Circle to Finite Line Force C1/1, Circle to Finite Line Force C4/1, Circle to Finite Line Force C3/1, Circle to Finite Line Force C2/1
  Circle to Finite Line Force C2/1 -> Sensing C1/1(S)
  Circle to Finite Line Force C1/1 -> Sensing C2/1(S)
  Add/1 -> Fn/1
  Sensing C1/1(Fn) -> Add/2
  Sensing C2/1(Fn) -> Add/1
  Sensing C4/1(Fn) -> Add/4
  Sensing C3/1(Fn) -> Add/3
  Circle to Finite Line Force C3/1 -> Sensing C3/1(S)
  Circle to Finite Line Force C4/1 -> Sensing C4/1(S)
  connections:
  Circle to Finite Line Force C2/LConn1 -- Transform C2/RConn1
  Transform C4/LConn1 -- Transform C3/LConn1 -- Box/RConn1 -- Transform C2/LConn1 -- Transform C1/LConn1
  Circle to Finite Line Force C1/LConn1 -- Transform C1/RConn1
  Circle to Finite Line Force C4/RConn1 -- Circle to Finite Line Force C3/RConn1 -- Bel/RConn1 -- Circle to Finite Line Force C2/RConn1 -- Circle to Finite Line Force C1/RConn1
  Circle to Finite Line Force C4/LConn1 -- Transform C4/RConn1
  Circle to Finite Line Force C3/LConn1 -- Transform C3/RConn1
